simulink model "tb_frames"  (R2026b)
undefined symbols (not defined in the file or in its folder): tb_frames_w
libraries: robotmobilelib x1
settings Model: Creator=aomar  LastModifiedBy=aomar

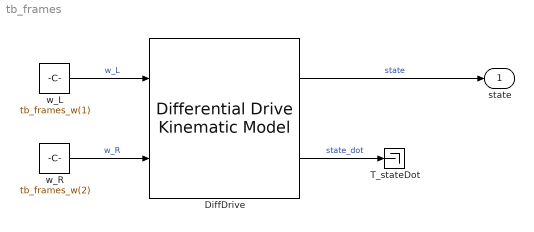
== system tb_frames ==
  DiffDrive : robotmobilelib/Differential Drive Kinematic Model  VehicleInputs=Wheel Speeds  WheelRadius=P.drive.gear.r_spr  WheelSpeedRange=[-inf inf]  TrackWidth=P.structure.geom.B  InitialState=tb_frames_x0  SimulateUsing=Interpreted execution
  T_stateDot : Terminator
  w_L : Constant  Value=tb_frames_w(1)
  w_R : Constant  Value=tb_frames_w(2)
  state : Outport
  wires:
  w_L/1 -> DiffDrive/1  "w_L"
  w_R/1 -> DiffDrive/2  "w_R"
  DiffDrive/1 -> state/1  "state"
  DiffDrive/2 -> T_stateDot/1  "state_dot"
